simulink model "My_gfm_pv_plus_sil"  (R2018b)
settings: Solver=ode45  StartTime=0.0  StopTime=30  RelTol=1e-3
PreLoadFcn:
  | lmodelDir = fileparts(get_param(bdroot,'FileName'));
  | 
  | load_system(fullfile(modelDir,'controls_element_lib.slx'));
  | load_system(fullfile(modelDir,'test_sequence_lib.slx'));
InitFcn:
  | close all;
  | clear all;
  | clc;
  | 
  | % frequency nominals
  | F_NOM = 60;
  | W_NOM = 2 * pi * F_NOM;
  | 
  | C_DC = 0.2; % Supercap: 0.5sec * 5MW
  | V_LVDC_NOM = 1000;
  | 
  | % base values relative to inverter
  | % --------------------------------
  | VLL_INV_NOM = 480;
  | P_INV_NOM = 1e6;
  | Q_INV_NOM = 0.5e6;
  | S_INV_NOM = sqrt(P_INV_NOM^2 + Q_INV_NOM^2);
  | 
  | I_INV_BASE = S_INV_NOM/(sqrt(3)*VLL_INV_NOM);
  | Z_INV_BASE = VLL_INV_NOM^2/S_INV_NOM;
  | L_INV_BASE = Z_INV_BASE / W_NOM;
  | C_INV_BASE = 1 / (Z_INV_BASE * W_NOM);
  | 
  | % nominal ratings for power system model
  | % --------------------------------------
  | INVERTER_COUNT = 100;
  | 
  | VLV_NOM = VLL_INV_NOM;
  | VMV_NOM = 35e3;
  | VHV_NOM = 230e3;
  | S_PLANT = INVERTER_COUNT * S_INV_NOM;
  | 
  | N_GSU = VHV_NOM/VMV_NOM;
  | N_MVT = VMV_NOM/VLV_NOM;
  | 
  | I_LV_BASE = S_PLANT/(sqrt(3)*VLV_NOM);
  | I_MV_BASE = S_PLANT/(sqrt(3)*VMV_NOM);
  | I_HV_BASE = S_PLANT/(sqrt(3)*VHV_NOM);
  | 
  | Z_LV_BASE = VLV_NOM^2/S_PLANT;
  | Z_MV_BASE = VMV_NOM^2/S_PLANT;
  | Z_HV_BASE = VHV_NOM^2/S_PLANT;
  | 
  | L_LV_BASE = Z_LV_BASE / W_NOM;
  | L_MV_BASE = Z_MV_BASE / W_NOM;
  | L_HV_BASE = Z_HV_BASE / W_NOM;
  | C_LV_BASE = 1 / (Z_LV_BASE * W_NOM);
  | C_MV_BASE = 1 / (Z_MV_BASE * W_NOM);
  | C_HV_BASE = 1 / (Z_HV_BASE * W_NOM);
libraries: test_sequence_lib x13, controls_element_lib x8
settings Model: SimulationMode=accelerator  Creator=halatrash  LastModifiedBy=ahhei
settings SolverCC: ZeroCrossAlgorithm=Adaptive
settings DataIOCC: ReturnWorkspaceOutputs=on
settings DebuggingCC: MaxConsecutiveZCsMsg=warning  IgnoredZcDiagnostic=none  UnconnectedInputMsg=none  UnconnectedOutputMsg=none  UnconnectedLineMsg=none
settings ModelReferenceCC: EnableRefExpFcnMdlSchedulingChecks=off
settings RTWCC: Description=Generic Real-Time Target

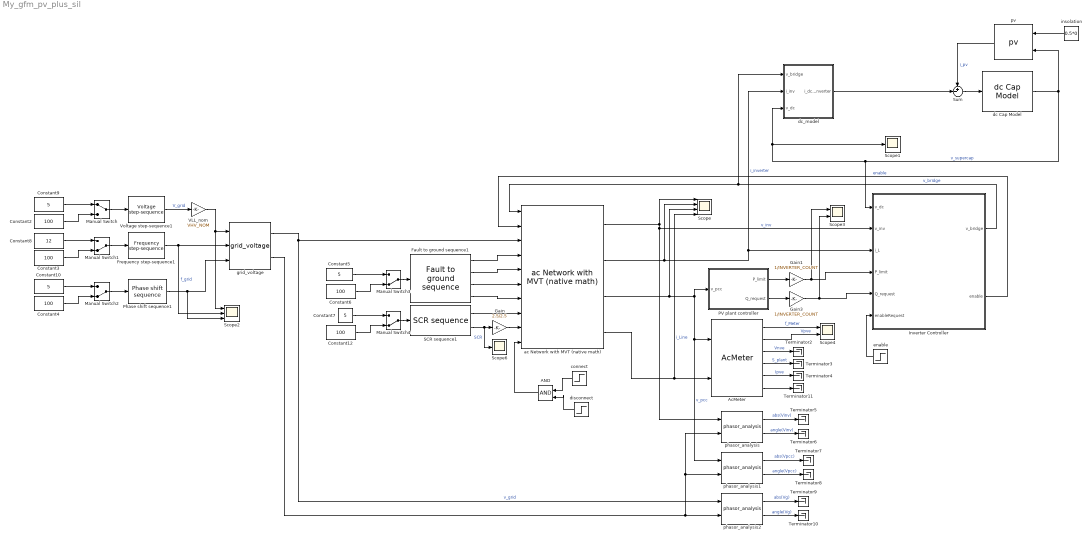
== system My_gfm_pv_plus_sil ==
  AND : Logic  IconShape=distinctive  AllPortsSameDT=off  OutDataTypeStr=boolean
  AcMeter : test_sequence_lib/AcMeter  VllRated=VHV_NOM
  Constant{5,7,9..10} (4 alike) : Constant  Value=5
  Constant{2..4,6,12} (5 alike) : Constant  Value=100
  Constant8 : Constant  Value=12
  Fault to ground sequence1 : test_sequence_lib/Fault to ground sequence  SystemSampleTime=-1
  Frequency step-sequence1 : test_sequence_lib/Frequency step-sequence  SystemSampleTime=-1
  Gain : Gain  Gain=2.5/2.5
  Gain1 : Gain  Gain=1/INVERTER_COUNT
  Gain3 : Gain  Gain=1/INVERTER_COUNT
  Inverter Controller : Subsystem
  Manual Switch : ManualSwitch
  Manual Switch{1..4} (4 alike) : ManualSwitch  CurrentSetting=0
  PV plant controller : Subsystem  AncestorBlock=controls_element_lib/PV plant controller
  Phase shift sequence1 : test_sequence_lib/Phase shift sequence  SystemSampleTime=-1
  SCR sequence1 : test_sequence_lib/SCR sequence  SystemSampleTime=-1
  Scope : Scope  NumInputPorts=4
  Scope1 : Scope
  Scope2 : Scope  NumInputPorts=3
  Scope3 : Scope  NumInputPorts=2
  Scope4 : Scope  NumInputPorts=2
  Scope6 : Scope
  Sum : Sum  Inputs=+-|
  Terminator{2..11} (10 alike) : Terminator
  VLL_nom : Gain  Gain=VHV_NOM
  Voltage step-sequence1 : test_sequence_lib/Voltage step-sequence  SystemSampleTime=-1
  ac Network with MVT (native math) : test_sequence_lib/ac Network with MVT (native math)  SystemSampleTime=-1
  connect : Step  Time=0  SampleTime=0
  dc Cap Model : test_sequence_lib/dc Cap Model  SystemSampleTime=-1
  dc_model : Subsystem  AncestorBlock=test_sequence_lib/dc_model
  disconnect : Step  Time=97  Before=1  After=0  SampleTime=0
  enable : Step  Time=2  SampleTime=0
  grid_voltage : test_sequence_lib/grid_voltage  SystemSampleTime=-1
  insolation : Constant  Value=0.5*0
  phasor_analysis : test_sequence_lib/phasor_analysis  SystemSampleTime=-1
  phasor_analysis1 : test_sequence_lib/phasor_analysis  SystemSampleTime=-1
  phasor_analysis2 : test_sequence_lib/phasor_analysis  SystemSampleTime=-1
  pv : test_sequence_lib/pv  VopenCircuit=1500  IshortCircuit=1000
  wires:
  ac Network with MVT (native math)/3 -> Scope/3, PV plant controller/1(v_pcc), phasor_analysis1/1, AcMeter/1  "v_pcc"
  Gain3/1 -> Scope3/2, Inverter Controller/5(Q_request)
  AcMeter/2 -> Scope4/2  "Vpve"
  phasor_analysis2/2 -> Terminator10/1  "angle(Vg)"
  phasor_analysis1/2 -> Terminator8/1  "angle(Vpcc)"
  AcMeter/5 -> Terminator4/1  "Ipve"
  phasor_analysis2/1 -> Terminator9/1  "abs(Vg)"
  Inverter Controller/1(v_bridge) -> ac Network with MVT (native math)/1, dc_model/1(v_bridge)  "v_bridge"
  phasor_analysis1/1 -> Terminator7/1  "abs(Vpcc)"
  grid_voltage/1 -> ac Network with MVT (native math)/3, phasor_analysis2/1  "v_grid"
  connect/1 -> AND/1
  dc Cap Model/1 -> pv/2, Scope1/1, dc_model/3(v_dc), Inverter Controller/1(v_dc)  "v_supercap"
  AcMeter/4 -> Terminator3/1  "S_plant"
  Phase shift sequence1/1 -> Scope2/3, grid_voltage/3
  Frequency step-sequence1/1 -> Scope2/2, grid_voltage/2  "f_grid"
  phasor_analysis/1 -> Terminator5/1  "abs(Vinv)"
  AcMeter/3 -> Terminator2/1  "Vnve"
  phasor_analysis/2 -> Terminator6/1  "angle(Vinv)"
  Sum/1 -> dc Cap Model/1
  ac Network with MVT (native math)/1 -> Scope/1, Inverter Controller/2(v_inv), phasor_analysis/1  "v_inv"
  AND/1 -> ac Network with MVT (native math)/10
  AcMeter/6 -> Terminator11/1
  Voltage step-sequence1/1 -> VLL_nom/1  "V_grid"
  grid_voltage/2 -> phasor_analysis1/2, phasor_analysis/2, phasor_analysis2/2
  disconnect/1 -> AND/2
  ac Network with MVT (native math)/2 -> Scope/2, Inverter Controller/3(i_L), dc_model/2(i_inv)  "i_inverter"
  PV plant controller/2(Q_request) -> Gain3/1
  ac Network with MVT (native math)/4 -> Scope/4, AcMeter/2  "i_Line"
  dc_model/1(i_dc_inverter) -> Sum/2
  Inverter Controller/2(enable) -> ac Network with MVT (native math)/2  "enable"
  VLL_nom/1 -> Scope2/1, grid_voltage/1
  enable/1 -> Inverter Controller/6(enableRequest)
  insolation/1 -> pv/1
  pv/1 -> Sum/1  "i_pv"
  PV plant controller/1(P_limit) -> Gain1/1
  Gain1/1 -> Scope3/1, Inverter Controller/4(P_limit)
  AcMeter/1 -> Scope4/1  "f_Meter"
  Constant10/1 -> Manual Switch2/1
  Constant9/1 -> Manual Switch/1
  Constant4/1 -> Manual Switch2/2
  Constant8/1 -> Manual Switch1/1
  Manual Switch1/1 -> Frequency step-sequence1/1
  Manual Switch2/1 -> Phase shift sequence1/1
  Manual Switch/1 -> Voltage step-sequence1/1
  Constant3/1 -> Manual Switch1/2
  Constant2/1 -> Manual Switch/2
  Constant12/1 -> Manual Switch4/2
  Constant6/1 -> Manual Switch3/2
  Manual Switch4/1 -> SCR sequence1/1
  Constant5/1 -> Manual Switch3/1
  Manual Switch3/1 -> Fault to ground sequence1/1
  Fault to ground sequence1/4 -> ac Network with MVT (native math)/7
  SCR sequence1/2 -> Scope6/1, Gain/1  "SCR"
  Fault to ground sequence1/1 -> ac Network with MVT (native math)/4
  SCR sequence1/1 -> ac Network with MVT (native math)/8
  Constant7/1 -> Manual Switch4/1
  Fault to ground sequence1/3 -> ac Network with MVT (native math)/6
  Fault to ground sequence1/2 -> ac Network with MVT (native math)/5
  Gain/1 -> ac Network with MVT (native math)/9

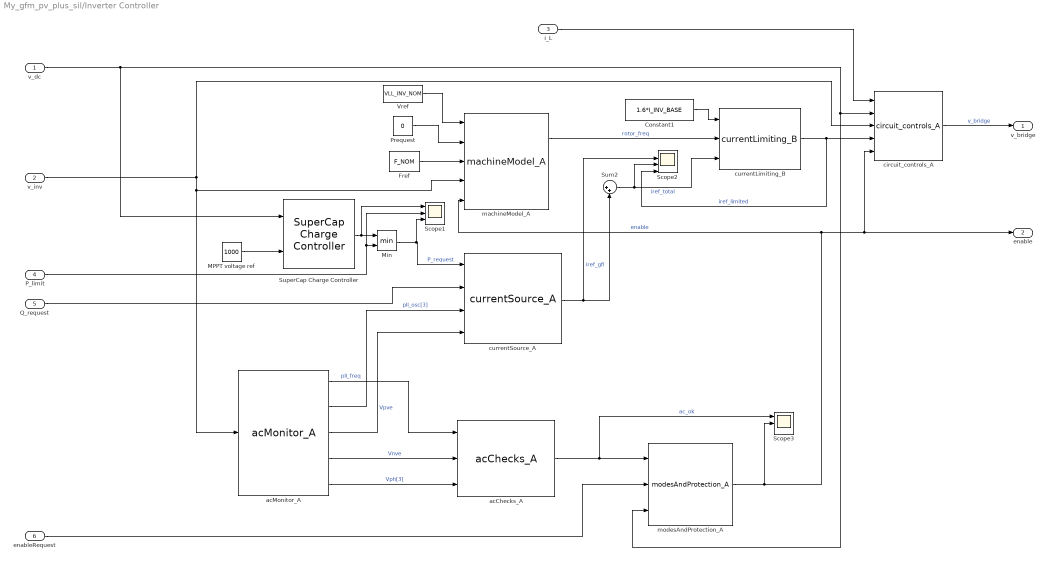
== system My_gfm_pv_plus_sil/Inverter Controller ==
  v_dc : Inport
  v_inv : Inport  Port=2
  i_L : Inport  Port=3
  P_limit : Inport  Port=4
  Q_request : Inport  Port=5
  enableRequest : Inport  Port=6
  Constant1 : Constant  Value=1.6*I_INV_BASE
  Fref : Constant  Value=F_NOM
  MPPT voltage ref : Constant  Value=1000
  Min : MinMax  Inputs=2
  Prequest : Constant  Value=0
  Scope1 : Scope  NumInputPorts=3
  Scope2 : Scope  NumInputPorts=4
  Scope3 : Scope  NumInputPorts=3
  Sum2 : Sum  Inputs=|++
  SuperCap Charge Controller : controls_element_lib/SuperCap Charge Controller  SystemSampleTime=-1
  Vref : Constant  Value=VLL_INV_NOM
  acChecks_A : controls_element_lib/acChecks_A  VllRated=VLL_INV_NOM  nominalFrequency=F_NOM  tRequalify=2  T_CNTL=1e-3
  acMonitor_A : controls_element_lib/acMonitor_A  VllRated=VLL_INV_NOM  nominalFrequency=F_NOM
  circuit_controls_A : controls_element_lib/circuit_controls_A  SystemSampleTime=-1
  currentLimiting_B : controls_element_lib/currentLimiting_B  IRated=I_INV_BASE  peakSoftLimit=2.6  peakHardLimit=3.6
  currentSource_A : controls_element_lib/currentSource_A  VllRated=VLL_INV_NOM  SRated=S_INV_NOM  nominalFrequency=F_NOM  Plimit=P_INV_NOM/S_INV_NOM  Qlimit=Q_INV_NOM/S_INV_NOM
  machineModel_A : controls_element_lib/machineModel_A  SRated=S_INV_NOM  VllRated=VLL_INV_NOM  nominalFrequency=F_NOM  inertialConstant=0.1  kDroop=0  kDamper=0.5  Xs=0.3  rs=0.08  Qlimit=0.5  wExciter=10
  modesAndProtection_A : controls_element_lib/modesAndProtection_A  dcOvervotlageThreshold=1800  dcUndervotlageThreshold=700  dcTripClearTimeout=0.2
  v_bridge : Outport  VectorParamsAs1DForOutWhenUnconnected=on
  enable : Outport  Port=2  VectorParamsAs1DForOutWhenUnconnected=on
  wires:
  Vref/1 -> machineModel_A/1
  Prequest/1 -> machineModel_A/2
  Fref/1 -> machineModel_A/3
  ? -> Scope2/1, Sum2/1  "iref_machine"
  currentLimiting_B/1 -> Scope2/4, circuit_controls_A/4  "iref_limited"
  v_inv/1 -> circuit_controls_A/3, acMonitor_A/1, machineModel_A/4
  currentSource_A/1 -> Scope2/2, Sum2/2  "iref_gfl"
  Sum2/1 -> Scope2/3, currentLimiting_B/3  "iref_total"
  acMonitor_A/2 -> currentSource_A/3  "pll_osc[3]"
  Q_request/1 -> currentSource_A/2
  acMonitor_A/4 -> acChecks_A/2  "Vnve"
  enableRequest/1 -> modesAndProtection_A/2
  modesAndProtection_A/1 -> Scope3/2, machineModel_A/5, circuit_controls_A/5, enable/1  "enable"
  Min/1 -> Scope1/3, currentSource_A/1  "P_request"
  acMonitor_A/3 -> currentSource_A/4  "Vpve"
  Constant1/1 -> currentLimiting_B/1
  acMonitor_A/5 -> acChecks_A/3  "Vph[3]"
  acChecks_A/1 -> Scope3/1, modesAndProtection_A/1  "ac_ok"
  acMonitor_A/1 -> acChecks_A/1  "pll_freq"
  circuit_controls_A/1 -> v_bridge/1  "v_bridge"
  v_dc/1 -> modesAndProtection_A/3, circuit_controls_A/2, SuperCap Charge Controller/1
  i_L/1 -> circuit_controls_A/1
  machineModel_A/1 -> currentLimiting_B/2  "rotor_freq"
  MPPT voltage ref/1 -> SuperCap Charge Controller/2
  SuperCap Charge Controller/1 -> Scope1/1, Min/1
  P_limit/1 -> Scope1/2, Min/2

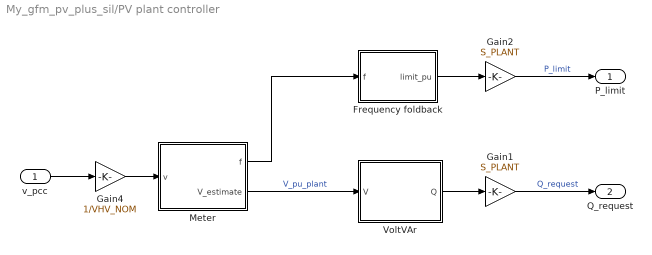
== system My_gfm_pv_plus_sil/PV plant controller ==
  v_pcc : Inport
  Frequency foldback : Subsystem
  Gain1 : Gain  Gain=S_PLANT
  Gain2 : Gain  Gain=S_PLANT
  Gain4 : Gain  Gain=1/VHV_NOM
  Meter : Subsystem
  VoltVAr : Subsystem
  P_limit : Outport  VectorParamsAs1DForOutWhenUnconnected=on
  Q_request : Outport  Port=2  VectorParamsAs1DForOutWhenUnconnected=on
  wires:
  Gain2/1 -> P_limit/1  "P_limit"
  Frequency foldback/1(limit_pu) -> Gain2/1
  Meter/1(f) -> Frequency foldback/1(f)
  v_pcc/1 -> Gain4/1
  Gain1/1 -> Q_request/1  "Q_request"
  Meter/2(V_estimate) -> VoltVAr/1(V)  "V_pu_plant"
  Gain4/1 -> Meter/1(v)
  VoltVAr/1(Q) -> Gain1/1

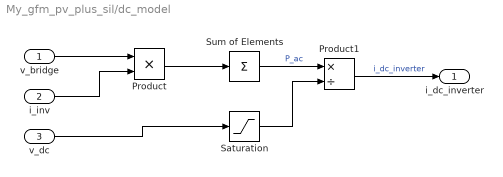
== system My_gfm_pv_plus_sil/dc_model ==
  v_bridge : Inport
  i_inv : Inport  Port=2
  v_dc : Inport  Port=3
  Product : Product
  Product1 : Product  Inputs=*/
  Saturation : Saturate  UpperLimit=inf  LowerLimit=10
  Sum of Elements : Sum  Inputs=+
  i_dc_inverter : Outport  VectorParamsAs1DForOutWhenUnconnected=on
  wires:
  Saturation/1 -> Product1/2
  v_bridge/1 -> Product/1
  Product1/1 -> i_dc_inverter/1  "i_dc_inverter"
  Product/1 -> Sum of Elements/1
  i_inv/1 -> Product/2
  Sum of Elements/1 -> Product1/1  "P_ac"
  v_dc/1 -> Saturation/1

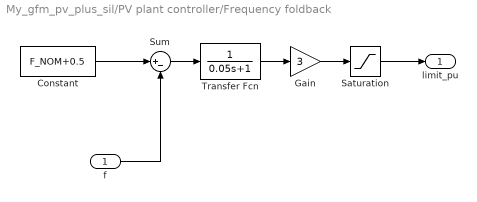
== system My_gfm_pv_plus_sil/PV plant controller/Frequency foldback ==
  f : Inport
  Constant : Constant  Value=F_NOM+0.5
  Gain : Gain  Gain=3
  Saturation : Saturate  UpperLimit=1  LowerLimit=0
  Sum : Sum  Inputs=|+-
  Transfer Fcn : TransferFcn  Denominator=[0.05 1]
  limit_pu : Outport  VectorParamsAs1DForOutWhenUnconnected=on
  wires:
  Saturation/1 -> limit_pu/1
  Constant/1 -> Sum/1
  Transfer Fcn/1 -> Gain/1
  Gain/1 -> Saturation/1
  f/1 -> Sum/2
  Sum/1 -> Transfer Fcn/1

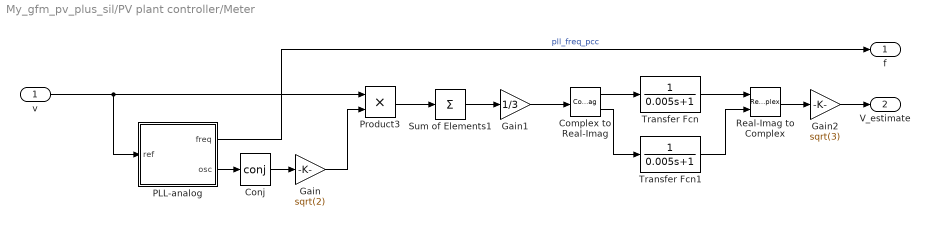
== system My_gfm_pv_plus_sil/PV plant controller/Meter ==
  v : Inport
  Complex to Real-Imag : ComplexToRealImag
  Conj : Math  Operator=conj  SaturateOnIntegerOverflow=on
  Gain : Gain  Gain=sqrt(2)
  Gain1 : Gain  Gain=1/3
  Gain2 : Gain  Gain=sqrt(3)
  PLL-analog : Subsystem
  Product3 : Product
  Real-Imag to Complex : RealImagToComplex
  Sum of Elements1 : Sum  Inputs=+
  Transfer Fcn : TransferFcn  Denominator=[0.005 1]
  Transfer Fcn1 : TransferFcn  Denominator=[0.005 1]
  f : Outport  VectorParamsAs1DForOutWhenUnconnected=on
  V_estimate : Outport  Port=2  VectorParamsAs1DForOutWhenUnconnected=on
  wires:
  PLL-analog/1(freq) -> f/1  "pll_freq_pcc"
  Gain2/1 -> V_estimate/1
  Gain1/1 -> Complex to Real-Imag/1
  Gain/1 -> Product3/2
  Real-Imag to Complex/1 -> Gain2/1
  Conj/1 -> Gain/1
  PLL-analog/2(osc) -> Conj/1
  Complex to Real-Imag/1 -> Transfer Fcn/1
  v/1 -> Product3/1, PLL-analog/1(ref)
  Complex to Real-Imag/2 -> Transfer Fcn1/1
  Product3/1 -> Sum of Elements1/1
  Transfer Fcn/1 -> Real-Imag to Complex/1
  Sum of Elements1/1 -> Gain1/1
  Transfer Fcn1/1 -> Real-Imag to Complex/2

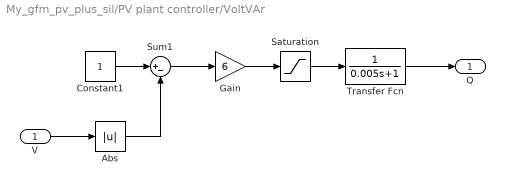
== system My_gfm_pv_plus_sil/PV plant controller/VoltVAr ==
  V : Inport
  Abs : Abs
  Constant1 : Constant
  Gain : Gain  Gain=6
  Saturation : Saturate
  Sum1 : Sum  Inputs=|+-
  Transfer Fcn : TransferFcn  Denominator=[0.005 1]
  Q : Outport  VectorParamsAs1DForOutWhenUnconnected=on
  wires:
  Transfer Fcn/1 -> Q/1
  Saturation/1 -> Transfer Fcn/1
  V/1 -> Abs/1
  Abs/1 -> Sum1/2
  Constant1/1 -> Sum1/1
  Sum1/1 -> Gain/1
  Gain/1 -> Saturation/1

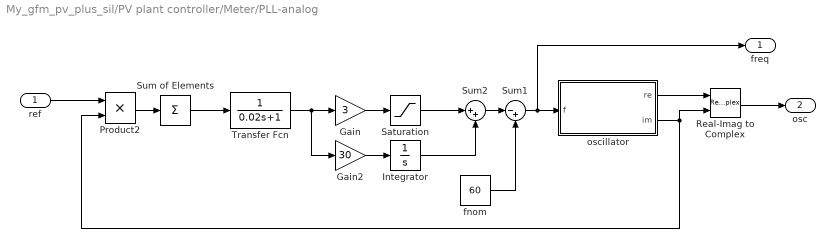
== system My_gfm_pv_plus_sil/PV plant controller/Meter/PLL-analog ==
  ref : Inport
  Gain : Gain  Gain=3
  Gain2 : Gain  Gain=30
  Integrator : Integrator  LimitOutput=on  UpperSaturationLimit=5  LowerSaturationLimit=-5
  Product2 : Product
  Real-Imag to Complex : RealImagToComplex
  Saturation : Saturate  UpperLimit=5  LowerLimit=-5
  Sum of Elements : Sum  Inputs=+
  Sum1 : Sum  Inputs=|-+
  Sum2 : Sum  Inputs=|++
  Transfer Fcn : TransferFcn  Denominator=[0.02 1]
  fnom : Constant  Value=60
  oscillator : Subsystem
  freq : Outport  VectorParamsAs1DForOutWhenUnconnected=on
  osc : Outport  Port=2  VectorParamsAs1DForOutWhenUnconnected=on
  wires:
  Gain2/1 -> Integrator/1
  Integrator/1 -> Sum2/2
  Sum2/1 -> Sum1/1
  fnom/1 -> Sum1/2
  Product2/1 -> Sum of Elements/1
  oscillator/2(im) -> Product2/2, Real-Imag to Complex/2
  Transfer Fcn/1 -> Gain/1, Gain2/1
  Saturation/1 -> Sum2/1
  Gain/1 -> Saturation/1
  Sum1/1 -> freq/1, oscillator/1(f)
  ref/1 -> Product2/1
  oscillator/1(re) -> Real-Imag to Complex/1
  Real-Imag to Complex/1 -> osc/1
  Sum of Elements/1 -> Transfer Fcn/1

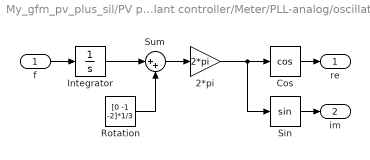
== system My_gfm_pv_plus_sil/PV plant controller/Meter/PLL-analog/oscillator ==
  f : Inport
  2*pi : Gain  Gain=2*pi
  Cos : Trigonometry  Operator=cos
  Integrator : Integrator
  Rotation : Constant  Value=[0 -1 -2]*1/3
  Sin : Trigonometry
  Sum : Sum  Inputs=|++
  re : Outport  VectorParamsAs1DForOutWhenUnconnected=on
  im : Outport  Port=2  VectorParamsAs1DForOutWhenUnconnected=on
  wires:
  2*pi/1 -> Sin/1, Cos/1
  f/1 -> Integrator/1
  Cos/1 -> re/1
  Sin/1 -> im/1
  Sum/1 -> 2*pi/1
  Integrator/1 -> Sum/1
  Rotation/1 -> Sum/2
